simulink model "LQG_linear_sim"  (R2026a)
settings: Solver=VariableStepAuto  StopTime=10
InitFcn:
  | seaDir=fileparts(get_param(bdroot,'FileName'));if isfile(fullfile(seaDir,'..','collaudo_simulink.m')),addpath(fullfile(seaDir,'..'));else,addpath(fullfile(seaDir,'..','..','File_di_Funzioni_Progetto-Accorpati'));end;collaudo_simulink(bdroot);
undefined symbols (not defined in the file): A, Aplant, B, Bplant, C, Cplant, Dplant, K, L, Nr, x0plant
libraries: dspstat3 x2
settings Model: Creator=rebec  LastModifiedBy=rebec

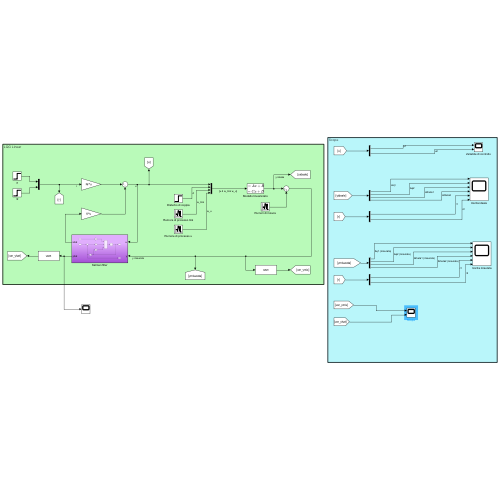
[thumbnail: Simulink's stored preview of the top-level diagram]
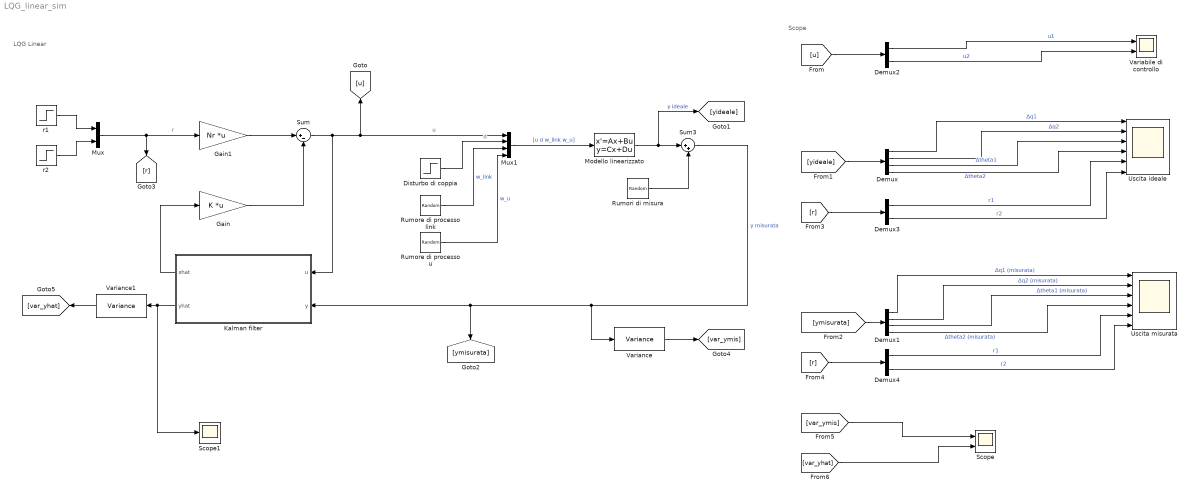
== system LQG_linear_sim ==
  note: Scope
  note: LQG Linear
  Demux : Demux
  Demux1 : Demux
  Demux2 : Demux  Outputs=2
  Demux3 : Demux  Outputs=2
  Demux4 : Demux  Outputs=2
  Disturbo di coppia : Step  Time=[1 1]  InitialValue=[0 0]  FinalValue=[0.5 0]  SampleTime=0
  Gain : Gain  Gain=K  Multiplication=Matrix(K*u)
  Gain1 : Gain  Gain=Nr  Multiplication=Matrix(K*u)
  Kalman filter : Subsystem
  Modello linearizzato : StateSpace  A=Aplant  B=Bplant  C=Cplant  D=Dplant  InitialCondition=x0plant
  Mux : Mux  Inputs=2
  Mux1 : Mux
  Rumore di processo link : RandomNumber  Mean=[0 0]  Variance=[0.01 0.01]  Seed=20260826  SampleTime=0.002
  Rumore di processo u : RandomNumber  Mean=[0 0]  Variance=[0.01 0.01]  Seed=20260826  SampleTime=0.002
  Rumori di misura : RandomNumber  Mean=[0 0 0 0]  Variance=[(0.05*pi/180)^2 (0.05*pi/180)^2 (0.05*pi/180)^2 (0.05*pi/180)^2]  Seed=20260826  SampleTime=0.002
  Scope : Scope  NumInputPorts=2
      settings: ActiveDisplayYMinimum=0.010186106284436241  ActiveDisplayYMaximum=0.011095969617899467  DataLoggingVariableName=ScopeData3
  Scope1 : Scope
      settings: ActiveDisplayYMinimum=-0.036853230362776712  ActiveDisplayYMaximum=0.3292427472168295  DataLoggingVariableName=ScopeData4
  Sum : Sum  Inputs=|+-
  Sum3 : Sum  Inputs=|++
  Uscita ideale : Scope  NumInputPorts=6
      settings: Title=Uscita ideale (LQG-LIN)  ActiveDisplayYMinimum=-0.094752290571448711  ActiveDisplayYMaximum=0.25948345010826868  YLabel=y (rad)
  Uscita misurata : Scope  NumInputPorts=6
      settings: Title=Uscita misurata (LQG-LIN)  ActiveDisplayYMinimum=-0.15271910419934975  ActiveDisplayYMaximum=0.19196102158094325  YLabel=y_m_i_s (rad)
  Variabile di controllo : Scope  NumInputPorts=2
      settings: Title=Variabili di controllo (LQG-LIN)  ActiveDisplayYMinimum=-2.6959450601265313  ActiveDisplayYMaximum=5.9059369724787079  YLabel=u (Nm)  DataLoggingVariableName=ScopeData2
  Variance : dspstat3/Variance  run=off  InputProcessing=Columns as channels (frame based)  reset_popup=None  directionMode=Each column  dimension=1  roiEnable=off  roiType=Rectangles  roiPortion=Entire ROI  roiOutput=Individual statistics for each ROI  roiFlag=off  roundingMode=Floor  overflowMode=off
  Variance1 : dspstat3/Variance  run=off  InputProcessing=Columns as channels (frame based)  reset_popup=None  directionMode=Each column  dimension=1  roiEnable=off  roiType=Rectangles  roiPortion=Entire ROI  roiOutput=Individual statistics for each ROI  roiFlag=off  roundingMode=Floor  overflowMode=off
  r1 : Step  FinalValue=5*pi/180  SampleTime=0
  r2 : Step  FinalValue=0  SampleTime=0
  wires:
  Demux/4 -> Uscita ideale/4  "Δtheta2"
  Demux2/1 -> Variabile di controllo/1  "u1"
  Demux1/1 -> Uscita misurata/1  "Δq1 (misurata)"
  r2/1 -> Mux/2
  Demux1/4 -> Uscita misurata/4  "Δtheta2 (misurata)"
  [r] -> Demux3/1
  Demux1/3 -> Uscita misurata/3  "Δtheta1 (misurata)"
  [u] -> Demux2/1
  [ymisurata] -> Demux1/1
  Demux3/1 -> Uscita ideale/5  "r1"
  Demux/1 -> Uscita ideale/1  "Δq1"
  Demux4/1 -> Uscita misurata/5  "r1"
  Demux1/2 -> Uscita misurata/2  "Δq2 (misurata)"
  Modello linearizzato/1 -> [yideale], Sum3/1  "y ideale"
  Sum3/1 -> Variance/1, Kalman filter/2(y), [ymisurata]  "y misurata"
  r1/1 -> Mux/1
  Gain1/1 -> Sum/1
  [yideale] -> Demux/1
  Demux2/2 -> Variabile di controllo/2  "u2"
  Demux/2 -> Uscita ideale/2  "Δq2"
  Demux/3 -> Uscita ideale/3  "Δtheta1"
  Demux3/2 -> Uscita ideale/6  "r2"
  Sum/1 -> Mux1/1, [u], Kalman filter/1(u)  "u"
  Demux4/2 -> Uscita misurata/6  "r2"
  Mux/1 -> [r], Gain1/1  "r"
  [r] -> Demux4/1
  Kalman filter/1(xhat) -> Gain/1
  Gain/1 -> Sum/2
  Rumore di processo u/1 -> Mux1/4  "w_u"
  Disturbo di coppia/1 -> Mux1/2  "d"
  Rumore di processo link/1 -> Mux1/3  "w_link"
  Mux1/1 -> Modello linearizzato/1  "[u d w_link w_u]"
  Rumori di misura/1 -> Sum3/2
  Kalman filter/2(yhat) -> Variance1/1, Scope1/1
  Variance/1 -> [var_ymis]
  Variance1/1 -> [var_yhat]
  [var_ymis] -> Scope/1
  [var_yhat] -> Scope/2

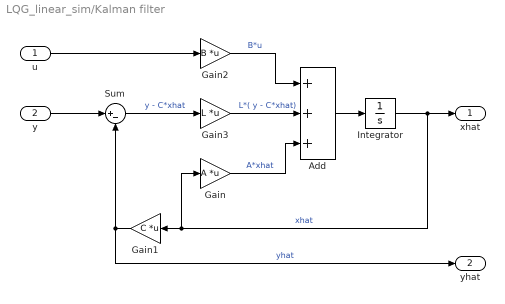
== system LQG_linear_sim/Kalman filter ==
  u : Inport
  y : Inport  Port=2
  Add : Sum  Inputs=+++
  Gain : Gain  Gain=A  Multiplication=Matrix(K*u)
  Gain1 : Gain  Gain=C  Multiplication=Matrix(K*u)
  Gain2 : Gain  Gain=B  Multiplication=Matrix(K*u)
  Gain3 : Gain  Gain=L  Multiplication=Matrix(K*u)
  Integrator : Integrator
  Sum : Sum  Inputs=|+-
  xhat : Outport
  yhat : Outport  Port=2
  wires:
  u/1 -> Gain2/1
  y/1 -> Sum/1
  Gain1/1 -> yhat/1, Sum/2  "yhat"
  Sum/1 -> Gain3/1  "y - C*xhat"
  Gain3/1 -> Add/2  "L*( y - C*xhat)"
  Gain2/1 -> Add/1  "B*u"
  Gain/1 -> Add/3  "A*xhat"
  Add/1 -> Integrator/1
  Integrator/1 -> Gain/1, Gain1/1, xhat/1  "xhat"
